simulink model "hrg_wa_a3_reference_manager"  (R2025a)
settings: Solver=FixedStepDiscrete  StartTime=0.0  StopTime=1.999  FixedStep=.001  RelTol=1e-3
InitFcn:
  | addpath(fileparts(fileparts(get_param(bdroot,'FileName'))));
model workspace (MAT data in the model file):
  a3_cfg.schema = 'A3-reference-covariance-v1'
  a3_cfg.reference_holdoff_s = 0.02
  a3_cfg.reanchor_period_s = 0.1
  a3_cfg.maximum_modal_direction_rate_rad_s = 30
  a3_cfg.phase_uncertainty_margin_rad = 0.02
  a3_cfg.recovery_guard_s = 0.02
  a3_cfg.noise_probe_max_abs_correlation = 0.1
  a3_cfg.noise_probe_correlation_lags = [1; 2; 3; 4]
  a3_cfg.kernel_impulse_samples = 16384
  a3_cfg.scope = '保留A2窗口、滤波与0.003rad预算；噪声协方差为白噪小扰动模型；重锚定保留全局初始参考；长缺测需外部参考'
  a3_cfg.sample_rate_Hz = 40000
  a3_cfg.carrier_Hz = 1000
  a3_cfg.duration_s = 2
  a3_cfg.regularizer_cutoff_Hz = 6000
  a3_cfg.washout_Hz = 1
  a3_cfg.demod_window_samples = 240
  a3_cfg.comparison_demod_window_samples = 240
  a3_cfg.reference_loop_bandwidth_Hz = 5
  a3_cfg.additional_phase_budget_rad = 0.2
  a3_cfg.frame_decimation = 40
  a3_cfg.warmup_s = 0.25
  a3_cfg.charge_scale_C = 1e-11
  a3_cfg.minimum_energy_normalized = 0.01
  a3_cfg.minimum_linearity = 0.98
  a3_cfg.angle_budget_rad = 0.003
  a3_cfg.sigma_multiplier = 3
  a3_cfg.calibration_Cs_relative_bound = 0.005
  a3_cfg.calibration_AFE_relative_bound = 0.005
  a3_cfg.calibration_false_reject_alpha = 0.001
  a3_cfg.noise_upper_alpha = 0.001
  a3_cfg.calibration_instrument_relative_sigma = 0.001
  a3_cfg.noise_probe_samples = 4096
  input_InitialGap = [0 0.001 0.002 0.003 0.004 0.005 0.006 0.007 0.008 0.009 0.01 0.011 ... (12000 elements, 2000x6)]
  input_LongGap = [0 0.001 0.002 0.003 0.004 0.005 0.006 0.007 0.008 0.009 0.01 0.011 ... (12000 elements, 2000x6)]
  input_Noise500u = [0 0.001 0.002 0.003 0.004 0.005 0.006 0.007 0.008 0.009 0.01 0.011 ... (12000 elements, 2000x6)]
  input_ShortGap = [0 0.001 0.002 0.003 0.004 0.005 0.006 0.007 0.008 0.009 0.01 0.011 ... (12000 elements, 2000x6)]
settings Model: Creator=11725  LastModifiedBy=11725

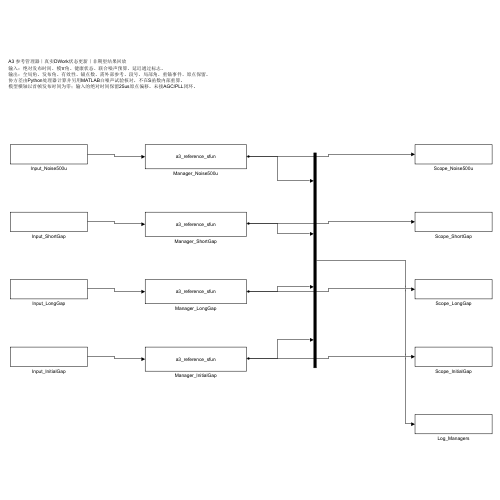
[thumbnail: Simulink's stored preview of the top-level diagram]
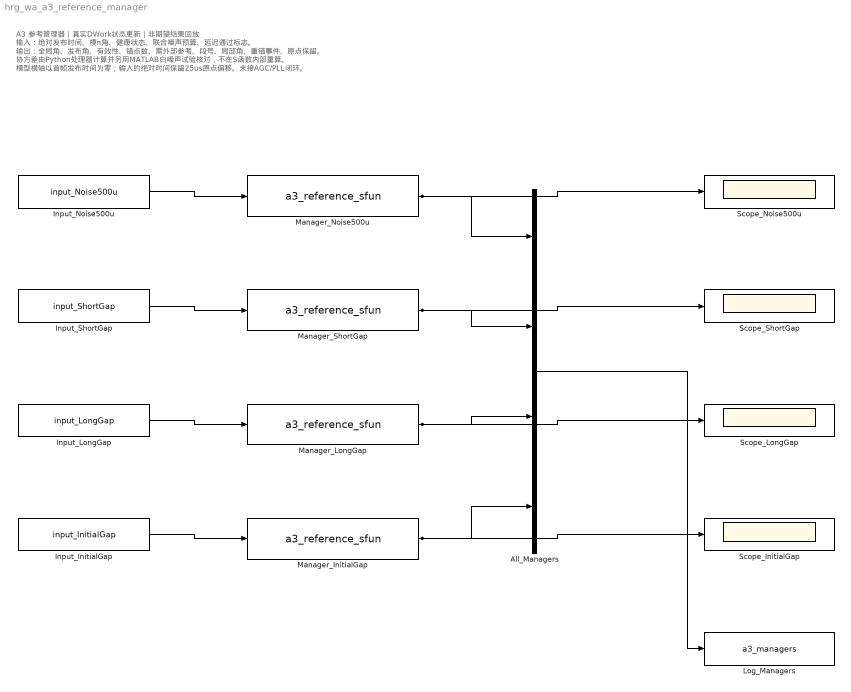
== system hrg_wa_a3_reference_manager ==
  note: A3 参考管理器｜真实DWork状态更新｜非期望结果回放
      | 输入：绝对发布时间、模π角、健康状态、联合噪声预算、延迟通过标志。
      | 输出：全局角、发布角、有效性、锚点数、需外部参考、段号、局部角、重锚事件、原点保留。
      | 协方差由Python处理器计算并另用MATLAB白噪声试验核对，不在S函数内部重算。
      | 模型横轴以首帧发布时间为零；输入的绝对时间保留25us原点偏移。未接AGC/PLL闭环。
  All_Managers : Mux
  Input_InitialGap : FromWorkspace  VariableName=input_InitialGap  SampleTime=.001  Interpolate=off  OutputAfterFinalValue=Holding final value
  Input_LongGap : FromWorkspace  VariableName=input_LongGap  SampleTime=.001  Interpolate=off  OutputAfterFinalValue=Holding final value
  Input_Noise500u : FromWorkspace  VariableName=input_Noise500u  SampleTime=.001  Interpolate=off  OutputAfterFinalValue=Holding final value
  Input_ShortGap : FromWorkspace  VariableName=input_ShortGap  SampleTime=.001  Interpolate=off  OutputAfterFinalValue=Holding final value
  Log_Managers : ToWorkspace  VariableName=a3_managers  SaveFormat=Timeseries  SampleTime=-1
  Manager_InitialGap : M-S-Function  FunctionName=a3_reference_sfun  Parameters=a3_cfg
  Manager_LongGap : M-S-Function  FunctionName=a3_reference_sfun  Parameters=a3_cfg
  Manager_Noise500u : M-S-Function  FunctionName=a3_reference_sfun  Parameters=a3_cfg
  Manager_ShortGap : M-S-Function  FunctionName=a3_reference_sfun  Parameters=a3_cfg
  Scope_InitialGap : Scope
  Scope_LongGap : Scope
  Scope_Noise500u : Scope
  Scope_ShortGap : Scope
  wires:
  Input_Noise500u/1 -> Manager_Noise500u/1
  Manager_Noise500u/1 -> Scope_Noise500u/1, All_Managers/1
  Input_ShortGap/1 -> Manager_ShortGap/1
  Manager_ShortGap/1 -> Scope_ShortGap/1, All_Managers/2
  Input_LongGap/1 -> Manager_LongGap/1
  Manager_LongGap/1 -> Scope_LongGap/1, All_Managers/3
  Input_InitialGap/1 -> Manager_InitialGap/1
  Manager_InitialGap/1 -> Scope_InitialGap/1, All_Managers/4
  All_Managers/1 -> Log_Managers/1
